simulink model "KneeReflexHuman"  (R2025a)
settings: Solver=ode15s  StartTime=0.0  StopTime=35  FixedStep=0.002  MaxStep=0.001  RelTol=1e-7  AbsTol=1e-9
PreLoadFcn:
  | activationTime=0.01;
  | deactivationTime=0.04;
  | sensoryPulse=2;
  | tapTorque=0;
  | eventTime=20;
  | pulseDuration=0.03;
  | torqueDuration=0.025;
libraries: SNS_Library x16
Description:
  | GUI-built Ia/Ib circuit with two compliant Gait2392 musculotendon blocks and a one-degree-of-freedom knee.
settings Model: Creator=Ben Bolen  LastModifiedBy=Ben Bolen
settings DataIOCC: SignalLogging=off

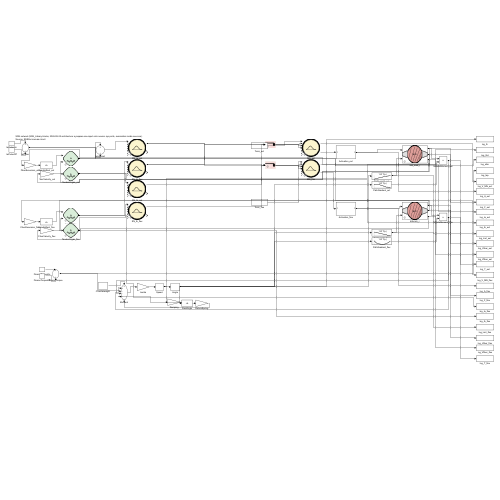
[thumbnail: Simulink's stored preview of the top-level diagram]
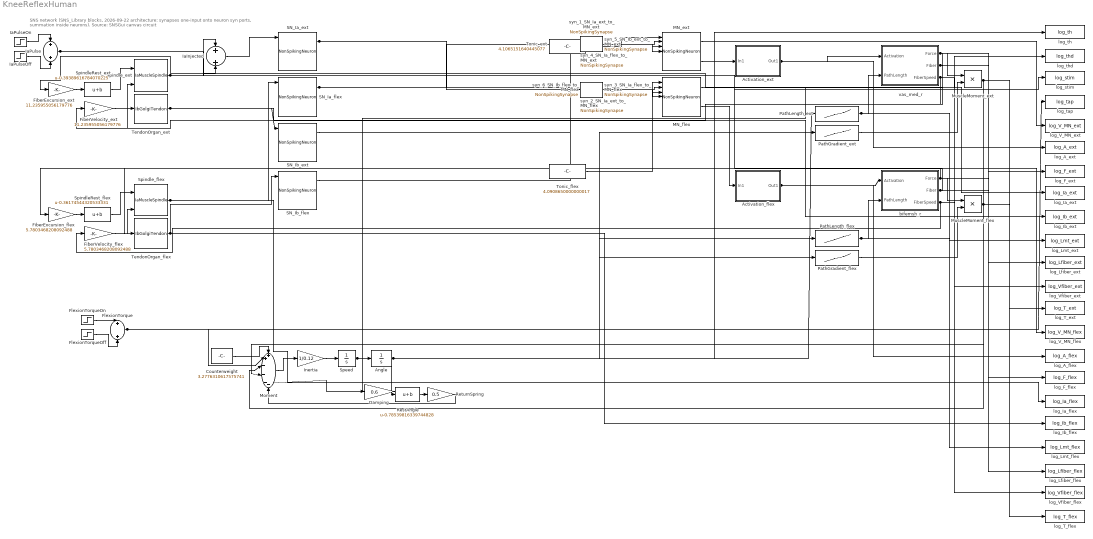
== system KneeReflexHuman ==
  note: SNS network (SNS_Library blocks, 2026-09-22 architecture: synapses one-input onto neuron syn ports, summation inside neurons).
      | Source: SNSGui canvas circuit
  Activation_ext : Subsystem
  Activation_flex : Subsystem
  Angle : Integrator  InitialCondition=0.78539816339744828
  Counterweight : Constant  Value=3.2776310617575741
  Damping : Gain  Gain=0.6
  FiberExcursion_ext : Gain  Gain=11.235955056179776
  FiberExcursion_flex : Gain  Gain=5.7803468208092488
  FiberVelocity_ext : Gain  Gain=11.235955056179776
  FiberVelocity_flex : Gain  Gain=5.7803468208092488
  FlexionTorque : Sum
  FlexionTorqueOff : Step  Time=eventTime+torqueDuration  After=-tapTorque  SampleTime=0
  FlexionTorqueOn : Step  Time=eventTime  After=tapTorque  SampleTime=0
  IaInjected : Sum
  IaPulse : Sum
  IaPulseOff : Step  Time=eventTime+pulseDuration  After=-sensoryPulse  SampleTime=0
  IaPulseOn : Step  Time=eventTime  After=sensoryPulse  SampleTime=0
  Inertia : Gain  Gain=1/0.12
  MN_ext : SNS_Library/NonSpikingNeuron  Vrest=-52  Gm=0.5  Cm=2.5  Thr=-45  Slope=10
  MN_flex : SNS_Library/NonSpikingNeuron  Vrest=-52  Gm=0.5  Cm=2.5  Thr=-45  Slope=10
  Moment : Sum  Inputs=++----
  MuscleMoment_ext : Product
  MuscleMoment_flex : Product
  PathGradient_ext : Lookup_n-D  NumberOfTableDimensions=1  BreakpointsForDimension1=[0 0.017453292519943295 0.034906585039886591 0.05235987755982989 0.069813170079773182 0.087266462599716474 0.10471975511965978 0.12217304763960307 0.13962634015954636 0.15707963267948966 0.17453292519943295 0.19198621771937624 0.20943951023931956 0.22689280275926285 0.24434609527920614 0.26179938779914941 0.27925268031909273 0.29670597283903605 0.31415926535897931 0.33161255787892263 0.3490658503988659 0.36651914291880922 0.38397243543875248 0.4014257279586958 0.41887902047863912 0.43633231299858238 0.4537856055185257 0.47123889803846897 0.48869219055841229 0.50614548307835561 0.52359877559829882 0.54105206811824214 0.55850536063818546 0.57595865315812877 0.59341194567807209 0.6108652381980153 0.62831853071795862 0.64577182323790194 0.66322511575784526 0.68067840827778847 0.69813170079773179 0.71558499331767511 0.73303828583761843 0.75049157835756175 0.76794487087750496 0.78539816339744828 0.8028514559173916 0.82030474843733492 0.83775804095727824 0.85521133347722145 0.87266462599716477 0.89011791851710809 0.90757121103705141 0.92502450355699462 0.94247779607693793 0.95993108859688125 0.97738438111682457 0.99483767363676789 1.0122909661567112 1.0297442586766545 1.0471975511965976 1.064650843716541 1.0821041362364843 1.0995574287564276 1.1170107212763709 1.1344640137963142 1.1519173063162575 1.1693705988362009 1.1868238913561442 1.2042771838760873 1.2217304763960306 1.2391837689159739 1.2566370614359172 1.2740903539558606 1.2915436464758039 1.3089969389957472 1.3264502315156905 1.3439035240356338 1.3613568165555769 1.3788101090755203 1.3962634015954636 1.4137166941154069 1.4311699866353502 1.4486232791552935 1.4660765716752369 1.4835298641951802 1.5009831567151235 1.5184364492350666 1.5358897417550099 1.5533430342749532 1.5707963267948966 1.5882496193148399 1.6057029118347832 1.6231562043547265 1.6406094968746698 1.6580627893946132]  Table=[0.046300541412696045 0.045945528146783335 0.04560618003400034 0.045291206631057568 0.045009747559742942 0.044771407689989967 0.044586287794695818 0.044465010200429353 0.044418738866694063 0.044459193231872661 0.044598655069569046 0.044792320710674169 0.044983515402986986 0.045166436487388571 0.045334488498150194 0.045480452453573142 0.045596644811568894 0.045675065799738478 0.045707536845315852 0.045685826873795007 0.045601767312865145 0.045488375392619018 0.0453804190740692 0.045272500382524589 0.045159280213405172 0.045035490671118006 0.044895946644946429 0.044735556564090159 0.04454933228582144 0.044332398083007075 0.044079998709690885 0.043802898012431105 0.043528262733400512 0.043256947497619311 0.042989173348334131 0.042725127360683068 0.042464964587145354 0.042208809868987306 0.041956759522132597 0.041708882905415239 0.041465223878729411 0.041220522162316059 0.040969567687275568 0.040712466844097947 0.040449332738228566 0.040180285292503316 0.039905451341858217 0.03962496472037294 0.039338966340718776 0.039047604266089025 0.038751033774698324 0.038449417416943923 0.038142925065329424 0.037831733957256544 0.037516028730797221 0.037196001453562624 0.036871851644790808 0.036543786290779014 0.036212019853789669 0.035876774274563865 0.035538278968577371 0.035198023590642488 0.034856945478862256 0.03451445183466019 0.034169952982176559 0.033822863200327721 0.033472601534141611 0.033118592585048387 0.032760267279801386 0.032397063617736394 0.032508073283476019 0.03247750725997104 0.032431791921784733 0.032371807186272486 0.032298273574261599 0.032211774977847177 0.032112778002968467 0.032001648442081303 0.031878665337946643 0.031744033021439806 0.031597891441606234 0.031437980227015702 0.0312622575156037 0.03107113358259856 0.030865597976765073 0.030649752356107715 0.030424658097017637 0.030190733110557224 0.02994839217600519 0.029698048006726905 0.029440112215267402 0.02917504524279816 0.028903309559376068 0.02862532065204686 0.028341496120541262 0.028052256309455396]  ExtrapMethod=Clip  InternalRulePriority=Speed  RndMeth=Simplest
  PathGradient_flex : Lookup_n-D  NumberOfTableDimensions=1  BreakpointsForDimension1=[0 0.017453292519943295 0.034906585039886591 0.05235987755982989 0.069813170079773182 0.087266462599716474 0.10471975511965978 0.12217304763960307 0.13962634015954636 0.15707963267948966 0.17453292519943295 0.19198621771937624 0.20943951023931956 0.22689280275926285 0.24434609527920614 0.26179938779914941 0.27925268031909273 0.29670597283903605 0.31415926535897931 0.33161255787892263 0.3490658503988659 0.36651914291880922 0.38397243543875248 0.4014257279586958 0.41887902047863912 0.43633231299858238 0.4537856055185257 0.47123889803846897 0.48869219055841229 0.50614548307835561 0.52359877559829882 0.54105206811824214 0.55850536063818546 0.57595865315812877 0.59341194567807209 0.6108652381980153 0.62831853071795862 0.64577182323790194 0.66322511575784526 0.68067840827778847 0.69813170079773179 0.71558499331767511 0.73303828583761843 0.75049157835756175 0.76794487087750496 0.78539816339744828 0.8028514559173916 0.82030474843733492 0.83775804095727824 0.85521133347722145 0.87266462599716477 0.89011791851710809 0.90757121103705141 0.92502450355699462 0.94247779607693793 0.95993108859688125 0.97738438111682457 0.99483767363676789 1.0122909661567112 1.0297442586766545 1.0471975511965976 1.064650843716541 1.0821041362364843 1.0995574287564276 1.1170107212763709 1.1344640137963142 1.1519173063162575 1.1693705988362009 1.1868238913561442 1.2042771838760873 1.2217304763960306 1.2391837689159739 1.2566370614359172 1.2740903539558606 1.2915436464758039 1.3089969389957472 1.3264502315156905 1.3439035240356338 1.3613568165555769 1.3788101090755203 1.3962634015954636 1.4137166941154069 1.4311699866353502 1.4486232791552935 1.4660765716752369 1.4835298641951802 1.5009831567151235 1.5184364492350666 1.5358897417550099 1.5533430342749532 1.5707963267948966 1.5882496193148399 1.6057029118347832 1.6231562043547265 1.6406094968746698 1.6580627893946132]  Table=[-0.020361084177321076 -0.02095432404287479 -0.021549948921287549 -0.022147893095183287 -0.022748075168790793 -0.023350397436992496 -0.023954745240616474 -0.024560986306975025 -0.025168970074611902 -0.025778527001181786 -0.026389467853347018 -0.026982156148773202 -0.027536386273640853 -0.028051147190922037 -0.028525485798045501 -0.028958501691153819 -0.029349341935763336 -0.029697195830473311 -0.030001289651172786 -0.030260881364096957 -0.030475255297092951 -0.030664144688230695 -0.030847730623721023 -0.031025982895034908 -0.031198868501991071 -0.031366351184743187 -0.031528390956651269 -0.031684943638144211 -0.031835960391693049 -0.031981387258029709 -0.032121164693761924 -0.032256849277144638 -0.032389988665417535 -0.032520500263503734 -0.032648294373979259 -0.032773273788839895 -0.032895333384571582 -0.033014359720642698 -0.033130230641547929 -0.033242814882547378 -0.033351971679259733 -0.033454060268764241 -0.0335453780438374 -0.033625689200947703 -0.03369476437945839 -0.033752380839864864 -0.033798322644897988 -0.033832380843261095 -0.033854353655739702 -0.033864046663389394 -0.033861272997474864 -0.03384585353079772 -0.03381761707001435 -0.033776400548507925 -0.033722049219339842 -0.033654416847766454 -0.033573365902766245 -0.033478767746981518 -0.033370502824436502 -0.033248460845351928 -0.033112540967333001 -0.032964251381959922 -0.03280509758262215 -0.032634983282771958 -0.032453816040338403 -0.032261507468146849 -0.032057973449924421 -0.031843134361701053 -0.031616915298350867 -0.031379246304984704 -0.031130062612869103 -0.030869260033517858 -0.030596740000038217 -0.030312454668946529 -0.03001636235322382 -0.029708427774943754 -0.029388622319715819 -0.029056924292337999 -0.028713319173009077 -0.028357799873408199 -0.027990366991891596 -0.027610663596923598 -0.027218353429907374 -0.026813481200552089 -0.026396101945645355 -0.025966281237410075 -0.025524095380485421 -0.025069631596368751 -0.024602988194139034 -0.02412427472627245 -0.023633612128355436 -0.0231311328415033 -0.022616980916300468 -0.022091312097095219 -0.021554293885504384 -0.021006105582016245]  ExtrapMethod=Clip  InternalRulePriority=Speed  RndMeth=Simplest
  PathLength_ext : Lookup_n-D  NumberOfTableDimensions=1  BreakpointsForDimension1=[0 0.017453292519943295 0.034906585039886591 0.05235987755982989 0.069813170079773182 0.087266462599716474 0.10471975511965978 0.12217304763960307 0.13962634015954636 0.15707963267948966 0.17453292519943295 0.19198621771937624 0.20943951023931956 0.22689280275926285 0.24434609527920614 0.26179938779914941 0.27925268031909273 0.29670597283903605 0.31415926535897931 0.33161255787892263 0.3490658503988659 0.36651914291880922 0.38397243543875248 0.4014257279586958 0.41887902047863912 0.43633231299858238 0.4537856055185257 0.47123889803846897 0.48869219055841229 0.50614548307835561 0.52359877559829882 0.54105206811824214 0.55850536063818546 0.57595865315812877 0.59341194567807209 0.6108652381980153 0.62831853071795862 0.64577182323790194 0.66322511575784526 0.68067840827778847 0.69813170079773179 0.71558499331767511 0.73303828583761843 0.75049157835756175 0.76794487087750496 0.78539816339744828 0.8028514559173916 0.82030474843733492 0.83775804095727824 0.85521133347722145 0.87266462599716477 0.89011791851710809 0.90757121103705141 0.92502450355699462 0.94247779607693793 0.95993108859688125 0.97738438111682457 0.99483767363676789 1.0122909661567112 1.0297442586766545 1.0471975511965976 1.064650843716541 1.0821041362364843 1.0995574287564276 1.1170107212763709 1.1344640137963142 1.1519173063162575 1.1693705988362009 1.1868238913561442 1.2042771838760873 1.2217304763960306 1.2391837689159739 1.2566370614359172 1.2740903539558606 1.2915436464758039 1.3089969389957472 1.3264502315156905 1.3439035240356338 1.3613568165555769 1.3788101090755203 1.3962634015954636 1.4137166941154069 1.4311699866353502 1.4486232791552935 1.4660765716752369 1.4835298641951802 1.5009831567151235 1.5184364492350666 1.5358897417550099 1.5533430342749532 1.5707963267948966 1.5882496193148399 1.6057029118347832 1.6231562043547265 1.6406094968746698 1.6580627893946132]  Table=[0.17226414023457803 0.17306912241670788 0.1738680327803396 0.17466122014122692 0.17544918902431589 0.17623260748310754 0.17701231549419177 0.17778933384389753 0.17856487341490523 0.17934034476994465 0.18011736791732169 0.18089745113888928 0.18168090068224443 0.18246762406431039 0.1832574203543533 0.18404996782905858 0.18484481449251688 0.18564137127820163 0.18643890774504843 0.18723655007529266 0.18803328117824838 0.18882818077722996 0.18962115663636275 0.19041225644225723 0.19120143416436042 0.19198855119117289 0.1927733776752531 0.19355559407317263 0.19433479286567448 0.19511048044259316 0.19588207913661326 0.19664900249551176 0.19741110599107001 0.19816844482247115 0.19892107891525168 0.19966907175352133 0.20041248980428711 0.20115140197454839 0.20188587909890082 0.202615993455526 0.20334181830858139 0.20406339673360424 0.20478064959247261 0.20549346867270485 0.2062017476771279 0.20690538234198108 0.20760427055673913 0.20829831248552194 0.20898741068995724 0.20967147025336369 0.2103503989061245 0.211024107152123 0.21169250839611231 0.21235551907189359 0.21301305877118049 0.21366505037302669 0.21431142017369864 0.21495209801687493 0.21558701742405872 0.21621611572508853 0.21683933418863893 0.21745662564317342 0.21806797220542951 0.21867335433892215 0.2192727421869049 0.21986609563416265 0.2204533643831465 0.22103448804408499 0.22160939623870357 0.22217800871717458 0.22274598949535074 0.22331311842427704 0.22387958026527199 0.22444511854181917 0.22500949070796325 0.22557246557043772 0.22613382107738966 0.22669334241891756 0.22725082039347982 0.22780605000157636 0.22835882923420606 0.22890894429032693 0.22945612978007696 0.2300001133427981 0.23054063134628333 0.2310774678055289 0.2316104557277896 0.23213943734621723 0.23266426215892685 0.23318478688379607 0.23370087543096607 0.23421239917621736 0.23471923783150911 0.23522127862909314 0.23571841607032532 0.23621055196811466]  ExtrapMethod=Clip  InternalRulePriority=Speed  RndMeth=Simplest
  PathLength_flex : Lookup_n-D  NumberOfTableDimensions=1  BreakpointsForDimension1=[0 0.017453292519943295 0.034906585039886591 0.05235987755982989 0.069813170079773182 0.087266462599716474 0.10471975511965978 0.12217304763960307 0.13962634015954636 0.15707963267948966 0.17453292519943295 0.19198621771937624 0.20943951023931956 0.22689280275926285 0.24434609527920614 0.26179938779914941 0.27925268031909273 0.29670597283903605 0.31415926535897931 0.33161255787892263 0.3490658503988659 0.36651914291880922 0.38397243543875248 0.4014257279586958 0.41887902047863912 0.43633231299858238 0.4537856055185257 0.47123889803846897 0.48869219055841229 0.50614548307835561 0.52359877559829882 0.54105206811824214 0.55850536063818546 0.57595865315812877 0.59341194567807209 0.6108652381980153 0.62831853071795862 0.64577182323790194 0.66322511575784526 0.68067840827778847 0.69813170079773179 0.71558499331767511 0.73303828583761843 0.75049157835756175 0.76794487087750496 0.78539816339744828 0.8028514559173916 0.82030474843733492 0.83775804095727824 0.85521133347722145 0.87266462599716477 0.89011791851710809 0.90757121103705141 0.92502450355699462 0.94247779607693793 0.95993108859688125 0.97738438111682457 0.99483767363676789 1.0122909661567112 1.0297442586766545 1.0471975511965976 1.064650843716541 1.0821041362364843 1.0995574287564276 1.1170107212763709 1.1344640137963142 1.1519173063162575 1.1693705988362009 1.1868238913561442 1.2042771838760873 1.2217304763960306 1.2391837689159739 1.2566370614359172 1.2740903539558606 1.2915436464758039 1.3089969389957472 1.3264502315156905 1.3439035240356338 1.3613568165555769 1.3788101090755203 1.3962634015954636 1.4137166941154069 1.4311699866353502 1.4486232791552935 1.4660765716752369 1.4835298641951802 1.5009831567151235 1.5184364492350666 1.5358897417550099 1.5533430342749532 1.5707963267948966 1.5882496193148399 1.6057029118347832 1.6231562043547265 1.6406094968746698 1.6580627893946132]  Table=[0.24625075890103157 0.2458902174580414 0.24551930112851292 0.24513796883726094 0.24474618079199639 0.24434389876245297 0.24393108637064406 0.2435077093925001 0.24307373607115063 0.24262913744213851 0.24217388767086862 0.24170807721638785 0.24123225649552227 0.2407471056410122 0.24025332191832333 0.23975161876020945 0.23924272489258069 0.23872738355168194 0.23820635179281544 0.23768039989104867 0.23715031083454793 0.23661676122560141 0.23607996111411669 0.23554000332275599 0.23499698122510049 0.23445098879845916 0.2339021206848379 0.23335047226005468 0.23279613971097904 0.23223922012087819 0.2316798115628457 0.23111800376309391 0.23055384991648156 0.22998739515578978 0.22941868611673941 0.22884777106551743 0.22827470003339995 0.22769952495841272 0.22712229983396864 0.22654308086441877 0.2259619266274511 0.22537891852748476 0.22479422229102369 0.22420802797125947 0.22362052968096371 0.22303192547848766 0.22244241725062483 0.22185221059228996 0.22126151468296998 0.2206705421599082 0.22007950898798781 0.21948863432628821 0.21889814039129254 0.21830825231673309 0.21771919801006898 0.21713120800559954 0.21654451531422519 0.21595935526987822 0.21537596537265757 0.2147945851287113 0.2142154558869237 0.21363881136446372 0.21306484964892342 0.21249376120230673 0.21192573813388765 0.21136097413128307 0.21079966438780465 0.21024200552599301 0.20968819551724283 0.20913843359743051 0.20859292017846437 0.2080518570165715 0.20751544789851614 0.20698389775873763 0.20645741231334186 0.20593619795044979 0.20542046161611893 0.20491041069581317 0.20440625289140499 0.20390819609370497 0.20341644825052965 0.20293121936125627 0.20245272761886318 0.2019811926777286 0.20151683332208922 0.20105986728396449 0.20061051105754235 0.20016897971023481 0.19973548669063176 0.19931024363360408 0.19889346016282591 0.19848534369100729 0.19808609921815051 0.19769592912816084 0.19731503298416755 0.19694360732292446]  ExtrapMethod=Clip  InternalRulePriority=Speed  RndMeth=Simplest
  RestAngle : Bias  Bias=-0.78539816339744828  SaturateOnIntegerOverflow=off
  ReturnSpring : Gain  Gain=0.5
  SN_Ia_ext : SNS_Library/NonSpikingNeuron  Vrest=-52  Gm=0.4  Cm=2  Thr=-55  Slope=1
  SN_Ia_flex : SNS_Library/NonSpikingNeuron  Vrest=-52  Gm=0.4  Cm=2  Thr=-55  Slope=1
  SN_Ib_ext : SNS_Library/NonSpikingNeuron  Vrest=-52  Gm=0.4  Cm=2  Thr=-55  Slope=1
  SN_Ib_flex : SNS_Library/NonSpikingNeuron  Vrest=-52  Gm=0.4  Cm=2  Thr=-55  Slope=1
  Speed : Integrator
  SpindleRest_ext : Bias  Bias=-0.39389616784070225  SaturateOnIntegerOverflow=off
  SpindleRest_flex : Bias  Bias=-0.36174544320533331  SaturateOnIntegerOverflow=off
  Spindle_ext : SNS_Library/IaMuscleSpindle  Imax=10  Wl=6  Wv=3
  Spindle_flex : SNS_Library/IaMuscleSpindle  Imax=10  Wl=6  Wv=3
  TendonOrgan_ext : SNS_Library/IbGolgiTendon  Imax=10  Kf=0.02
  TendonOrgan_flex : SNS_Library/IbGolgiTendon  Imax=10  Kf=0.022200000000000001
  Tonic_ext : Constant  Value=4.1065151640445077
  Tonic_flex : Constant  Value=4.0908650000000017
  bifemsh_r : Subsystem  mask(Gait2392 Thelen2003 biological muscle){}
      mask help: Elastic tendon, active and passive fibers, and constant-height pennation driven by Gait2392 parameters.
      mask Display:
      | patch([-0.58 -0.5558 -0.5317 -0.5075 -0.4833 -0.4592 -0.435 -0.4108 -0.3867 -0.3625 -0.3383 -0.3142 -0.29 -0.2658 -0.2417 -0.2175 -0.1933 -0.1692 -0.145 -0.1208 -0.09667 -0.0725 -0.04833 -0.02417 0 0.02417 0.04833 0.0725 0.09667 0.1208 0.145 0.1692 0.1933 0.2175 0.2417 0.2658 0.29 0.3142 0.3383 0.3625 0.3867 0.4108 0.435 0.4592 0.4833 0.5075 0.5317 0.5558 0.58 0.58 0.5558 0.5317 0.5075 0.4833 0.4592 0.435 0.4108 0.3867 0.3625 0.3383 0.3142 0.29 0.2658 0.2417 0.2175 0.1933 0.1692 0.145 0.1208 0.09667 0.0725 0.04833 0.02417 0 -0.02417 -0.04833 -0.0725 -0.09667 -0.1208 -0.145 -0.1692 -0.1933 -0.2175 -0.2417 -0.2658 -0.29 -0.3142 -0.3383 -0.3625 -0.3867 -0.4108 -0.435 -0.4592 -0.4833 -0.5075 -0.5317 -0.5558 -0.58], [0.022 0.07714 0.1114 0.1399 0.1647 0.1868 0.2067 0.2249 0.2414 0.2565 0.2703 0.2829 0.2943 0.3047 0.314 0.3224 0.3298 0.3362 0.3418 0.3465 0.3503 0.3532 0.3553 0.3566 0.357 0.3566 0.3553 0.3532 0.3503 0.3465 0.3418 0.3362 0.3298 0.3224 0.314 0.3047 0.2943 0.2829 0.2703 0.2565 0.2414 0.2249 0.2067 0.1868 0.1647 0.1399 0.1114 0.07714 0.022 0.022 -0.07714 -0.1114 -0.1399 -0.1647 -0.1868 -0.2067 -0.2249 -0.2414 -0.2565 -0.2703 -0.2829 -0.2943 -0.3047 -0.314 -0.3224 -0.3298 -0.3362 -0.3418 -0.3465 -0.3503 -0.3532 -0.3553 -0.3566 -0.357 -0.3566 -0.3553 -0.3532 -0.3503 -0.3465 -0.3418 -0.3362 -0.3298 -0.3224 -0.314 -0.3047 -0.2943 -0.2829 -0.2703 -0.2565 -0.2414 -0.2249 -0.2067 -0.1868 -0.1647 -0.1399 -0.1114 -0.07714 0.022], [0 0 0]);
      | patch([-0.58 -0.5558 -0.5317 -0.5075 -0.4833 -0.4592 -0.435 -0.4108 -0.3867 -0.3625 -0.3383 -0.3142 -0.29 -0.2658 -0.2417 -0.2175 -0.1933 -0.1692 -0.145 -0.1208 -0.09667 -0.0725 -0.04833 -0.02417 0 0.02417 0.04833 0.0725 0.09667 0.1208 0.145 0.1692 0.1933 0.2175 0.2417 0.2658 0.29 0.3142 0.3383 0.3625 0.3867 0.4108 0.435 0.4592 0.4833 0.5075 0.5317 0.5558 0.58 0.58 0.5558 0.5317 0.5075 0.4833 0.4592 0.435 0.4108 0.3867 0.3625 0.3383 0.3142 0.29 0.2658 0.2417 0.2175 0.1933 0.1692 0.145 0.1208 0.09667 0.0725 0.04833 0.02417 0 -0.02417 -0.04833 -0.0725 -0.09667 -0.1208 -0.145 -0.1692 -0.1933 -0.2175 -0.2417 -0.2658 -0.29 -0.3142 -0.3383 -0.3625 -0.3867 -0.4108 -0.435 -0.4592 -0.4833 -0.5075 -0.5317 -0.5558 -0.58], [0 0.05514 0.08943 0.1179 0.1427 0.1648 0.1847 0.2029 0.2194 0.2345 0.2483 0.2609 0.2723 0.2827 0.292 0.3004 0.3078 0.3142 0.3198 0.3245 0.3283 0.3312 0.3333 0.3346 0.335 0.3346 0.3333 0.3312 0.3283 0.3245 0.3198 0.3142 0.3078 0.3004 0.292 0.2827 0.2723 0.2609 0.2483 0.2345 0.2194 0.2029 0.1847 0.1648 0.1427 0.1179 0.08943 0.05514 0 -0 -0.05514 -0.08943 -0.1179 -0.1427 -0.1648 -0.1847 -0.2029 -0.2194 -0.2345 -0.2483 -0.2609 -0.2723 -0.2827 -0.292 -0.3004 -0.3078 -0.3142 -0.3198 -0.3245 -0.3283 -0.3312 -0.3333 -0.3346 -0.335 -0.3346 -0.3333 -0.3312 -0.3283 -0.3245 -0.3198 -0.3142 -0.3078 -0.3004 -0.292 -0.2827 -0.2723 -0.2609 -0.2483 -0.2345 -0.2194 -0.2029 -0.1847 -0.1648 -0.1427 -0.1179 -0.08943 -0.05514 -0], [0.87 0.62 0.6]);
      | color('black');
      | plot([-0.46 -0.2855], [-0.1476 0.2469]);
      | plot([-0.305 -0.02282], [-0.2388 0.3012]);
      | plot([-0.15 0.1889], [-0.2868 0.2781]);
      | plot([0.005 0.3612], [-0.3015 0.2117]);
      | plot([0.16 0.4965], [-0.2848 0.1166]);
      | plot([0.315 0.52], [-0.2344 0.09333]);
      | plot([0.47 0.52], [-0.1396 0.09333]);
      | patch([0.58 0.95 0.95 0.58], [-0.148 -0.068 0.068 0.148], [0 0 0]);
      | patch([0.58 0.95 0.95 0.58], [-0.13 -0.05 0.05 0.13], [0.88 0.88 0.88]);
      | patch([-0.58 -0.95 -0.95 -0.58], [-0.148 -0.068 0.068 0.148], [0 0 0]);
      | patch([-0.58 -0.95 -0.95 -0.58], [-0.13 -0.05 0.05 0.13], [0.88 0.88 0.88]);
      | disp('BIO');
  log_A_ext : ToWorkspace  VariableName=log_A_ext  SaveFormat=Timeseries  SampleTime=-1
  log_A_flex : ToWorkspace  VariableName=log_A_flex  SaveFormat=Timeseries  SampleTime=-1
  log_F_ext : ToWorkspace  VariableName=log_F_ext  SaveFormat=Timeseries  SampleTime=-1
  log_F_flex : ToWorkspace  VariableName=log_F_flex  SaveFormat=Timeseries  SampleTime=-1
  log_Ia_ext : ToWorkspace  VariableName=log_Ia_ext  SaveFormat=Timeseries  SampleTime=-1
  log_Ia_flex : ToWorkspace  VariableName=log_Ia_flex  SaveFormat=Timeseries  SampleTime=-1
  log_Ib_ext : ToWorkspace  VariableName=log_Ib_ext  SaveFormat=Timeseries  SampleTime=-1
  log_Ib_flex : ToWorkspace  VariableName=log_Ib_flex  SaveFormat=Timeseries  SampleTime=-1
  log_Lfiber_ext : ToWorkspace  VariableName=log_Lfiber_ext  SaveFormat=Timeseries  SampleTime=-1
  log_Lfiber_flex : ToWorkspace  VariableName=log_Lfiber_flex  SaveFormat=Timeseries  SampleTime=-1
  log_Lmt_ext : ToWorkspace  VariableName=log_Lmt_ext  SaveFormat=Timeseries  SampleTime=-1
  log_Lmt_flex : ToWorkspace  VariableName=log_Lmt_flex  SaveFormat=Timeseries  SampleTime=-1
  log_T_ext : ToWorkspace  VariableName=log_T_ext  SaveFormat=Timeseries  SampleTime=-1
  log_T_flex : ToWorkspace  VariableName=log_T_flex  SaveFormat=Timeseries  SampleTime=-1
  log_V_MN_ext : ToWorkspace  VariableName=log_V_MN_ext  SaveFormat=Timeseries  SampleTime=-1
  log_V_MN_flex : ToWorkspace  VariableName=log_V_MN_flex  SaveFormat=Timeseries  SampleTime=-1
  log_Vfiber_ext : ToWorkspace  VariableName=log_Vfiber_ext  SaveFormat=Timeseries  SampleTime=-1
  log_Vfiber_flex : ToWorkspace  VariableName=log_Vfiber_flex  SaveFormat=Timeseries  SampleTime=-1
  log_stim : ToWorkspace  VariableName=log_stim  SaveFormat=Timeseries  SampleTime=-1
  log_tap : ToWorkspace  VariableName=log_tap  SaveFormat=Timeseries  SampleTime=-1
  log_th : ToWorkspace  VariableName=log_th  SaveFormat=Timeseries  SampleTime=-1
  log_thd : ToWorkspace  VariableName=log_thd  SaveFormat=Timeseries  SampleTime=-1
  syn_1_SN_Ia_ext_to_MN_ext : SNS_Library/NonSpikingSynapse  gmax=0.009  Esyn=0  ThrPre=-45  SlopePre=10
  syn_2_SN_Ia_ext_to_MN_flex : SNS_Library/NonSpikingSynapse  gmax=0.0075  Esyn=-72  ThrPre=-45  SlopePre=10
  syn_3_SN_Ia_flex_to_MN_flex : SNS_Library/NonSpikingSynapse  gmax=0.009  Esyn=0  ThrPre=-45  SlopePre=10
  syn_4_SN_Ia_flex_to_MN_ext : SNS_Library/NonSpikingSynapse  gmax=0.0075  Esyn=-72  ThrPre=-45  SlopePre=10
  syn_5_SN_Ib_ext_to_MN_ext : SNS_Library/NonSpikingSynapse  gmax=0.01  Esyn=-72  ThrPre=-45  SlopePre=10
  syn_6_SN_Ib_flex_to_MN_flex : SNS_Library/NonSpikingSynapse  gmax=0.01  Esyn=-72  ThrPre=-45  SlopePre=10
  vas_med_r : Subsystem  mask(Gait2392 Thelen2003 biological muscle){}
      mask help: Elastic tendon, active and passive fibers, and constant-height pennation driven by Gait2392 parameters.
      mask Display:
      | patch([-0.58 -0.5558 -0.5317 -0.5075 -0.4833 -0.4592 -0.435 -0.4108 -0.3867 -0.3625 -0.3383 -0.3142 -0.29 -0.2658 -0.2417 -0.2175 -0.1933 -0.1692 -0.145 -0.1208 -0.09667 -0.0725 -0.04833 -0.02417 0 0.02417 0.04833 0.0725 0.09667 0.1208 0.145 0.1692 0.1933 0.2175 0.2417 0.2658 0.29 0.3142 0.3383 0.3625 0.3867 0.4108 0.435 0.4592 0.4833 0.5075 0.5317 0.5558 0.58 0.58 0.5558 0.5317 0.5075 0.4833 0.4592 0.435 0.4108 0.3867 0.3625 0.3383 0.3142 0.29 0.2658 0.2417 0.2175 0.1933 0.1692 0.145 0.1208 0.09667 0.0725 0.04833 0.02417 0 -0.02417 -0.04833 -0.0725 -0.09667 -0.1208 -0.145 -0.1692 -0.1933 -0.2175 -0.2417 -0.2658 -0.29 -0.3142 -0.3383 -0.3625 -0.3867 -0.4108 -0.435 -0.4592 -0.4833 -0.5075 -0.5317 -0.5558 -0.58], [0.022 0.07714 0.1114 0.1399 0.1647 0.1868 0.2067 0.2249 0.2414 0.2565 0.2703 0.2829 0.2943 0.3047 0.314 0.3224 0.3298 0.3362 0.3418 0.3465 0.3503 0.3532 0.3553 0.3566 0.357 0.3566 0.3553 0.3532 0.3503 0.3465 0.3418 0.3362 0.3298 0.3224 0.314 0.3047 0.2943 0.2829 0.2703 0.2565 0.2414 0.2249 0.2067 0.1868 0.1647 0.1399 0.1114 0.07714 0.022 0.022 -0.07714 -0.1114 -0.1399 -0.1647 -0.1868 -0.2067 -0.2249 -0.2414 -0.2565 -0.2703 -0.2829 -0.2943 -0.3047 -0.314 -0.3224 -0.3298 -0.3362 -0.3418 -0.3465 -0.3503 -0.3532 -0.3553 -0.3566 -0.357 -0.3566 -0.3553 -0.3532 -0.3503 -0.3465 -0.3418 -0.3362 -0.3298 -0.3224 -0.314 -0.3047 -0.2943 -0.2829 -0.2703 -0.2565 -0.2414 -0.2249 -0.2067 -0.1868 -0.1647 -0.1399 -0.1114 -0.07714 0.022], [0 0 0]);
      | patch([-0.58 -0.5558 -0.5317 -0.5075 -0.4833 -0.4592 -0.435 -0.4108 -0.3867 -0.3625 -0.3383 -0.3142 -0.29 -0.2658 -0.2417 -0.2175 -0.1933 -0.1692 -0.145 -0.1208 -0.09667 -0.0725 -0.04833 -0.02417 0 0.02417 0.04833 0.0725 0.09667 0.1208 0.145 0.1692 0.1933 0.2175 0.2417 0.2658 0.29 0.3142 0.3383 0.3625 0.3867 0.4108 0.435 0.4592 0.4833 0.5075 0.5317 0.5558 0.58 0.58 0.5558 0.5317 0.5075 0.4833 0.4592 0.435 0.4108 0.3867 0.3625 0.3383 0.3142 0.29 0.2658 0.2417 0.2175 0.1933 0.1692 0.145 0.1208 0.09667 0.0725 0.04833 0.02417 0 -0.02417 -0.04833 -0.0725 -0.09667 -0.1208 -0.145 -0.1692 -0.1933 -0.2175 -0.2417 -0.2658 -0.29 -0.3142 -0.3383 -0.3625 -0.3867 -0.4108 -0.435 -0.4592 -0.4833 -0.5075 -0.5317 -0.5558 -0.58], [0 0.05514 0.08943 0.1179 0.1427 0.1648 0.1847 0.2029 0.2194 0.2345 0.2483 0.2609 0.2723 0.2827 0.292 0.3004 0.3078 0.3142 0.3198 0.3245 0.3283 0.3312 0.3333 0.3346 0.335 0.3346 0.3333 0.3312 0.3283 0.3245 0.3198 0.3142 0.3078 0.3004 0.292 0.2827 0.2723 0.2609 0.2483 0.2345 0.2194 0.2029 0.1847 0.1648 0.1427 0.1179 0.08943 0.05514 0 -0 -0.05514 -0.08943 -0.1179 -0.1427 -0.1648 -0.1847 -0.2029 -0.2194 -0.2345 -0.2483 -0.2609 -0.2723 -0.2827 -0.292 -0.3004 -0.3078 -0.3142 -0.3198 -0.3245 -0.3283 -0.3312 -0.3333 -0.3346 -0.335 -0.3346 -0.3333 -0.3312 -0.3283 -0.3245 -0.3198 -0.3142 -0.3078 -0.3004 -0.292 -0.2827 -0.2723 -0.2609 -0.2483 -0.2345 -0.2194 -0.2029 -0.1847 -0.1648 -0.1427 -0.1179 -0.08943 -0.05514 -0], [0.87 0.62 0.6]);
      | color('black');
      | plot([-0.46 -0.2855], [-0.1476 0.2469]);
      | plot([-0.305 -0.02282], [-0.2388 0.3012]);
      | plot([-0.15 0.1889], [-0.2868 0.2781]);
      | plot([0.005 0.3612], [-0.3015 0.2117]);
      | plot([0.16 0.4965], [-0.2848 0.1166]);
      | plot([0.315 0.52], [-0.2344 0.09333]);
      | plot([0.47 0.52], [-0.1396 0.09333]);
      | patch([0.58 0.95 0.95 0.58], [-0.148 -0.068 0.068 0.148], [0 0 0]);
      | patch([0.58 0.95 0.95 0.58], [-0.13 -0.05 0.05 0.13], [0.88 0.88 0.88]);
      | patch([-0.58 -0.95 -0.95 -0.58], [-0.148 -0.068 0.068 0.148], [0 0 0]);
      | patch([-0.58 -0.95 -0.95 -0.58], [-0.13 -0.05 0.05 0.13], [0.88 0.88 0.88]);
      | disp('BIO');
  wires:
  syn_1_SN_Ia_ext_to_MN_ext/1 -> MN_ext/2
  syn_4_SN_Ia_flex_to_MN_ext/1 -> MN_ext/3
  syn_5_SN_Ib_ext_to_MN_ext/1 -> MN_ext/4
  syn_2_SN_Ia_ext_to_MN_flex/1 -> MN_flex/2
  syn_3_SN_Ia_flex_to_MN_flex/1 -> MN_flex/3
  syn_6_SN_Ib_flex_to_MN_flex/1 -> MN_flex/4
  SN_Ia_ext/1 -> syn_1_SN_Ia_ext_to_MN_ext/1, syn_2_SN_Ia_ext_to_MN_flex/1
  SN_Ia_flex/1 -> syn_3_SN_Ia_flex_to_MN_flex/1, syn_4_SN_Ia_flex_to_MN_ext/1
  SN_Ib_ext/1 -> syn_5_SN_Ib_ext_to_MN_ext/1
  SN_Ib_flex/1 -> syn_6_SN_Ib_flex_to_MN_flex/1
  Moment/1 -> Inertia/1
  Inertia/1 -> Speed/1
  Speed/1 -> Angle/1, Damping/1, log_thd/1
  Angle/1 -> RestAngle/1, PathLength_ext/1, PathGradient_ext/1, PathLength_flex/1, PathGradient_flex/1, log_th/1
  RestAngle/1 -> ReturnSpring/1
  Counterweight/1 -> Moment/1
  Damping/1 -> Moment/5
  ReturnSpring/1 -> Moment/6
  IaPulseOn/1 -> IaPulse/1
  IaPulseOff/1 -> IaPulse/2
  FlexionTorqueOn/1 -> FlexionTorque/1
  FlexionTorqueOff/1 -> FlexionTorque/2
  FlexionTorque/1 -> Moment/2, log_tap/1
  MN_ext/2 -> Activation_ext/1(In1)
  Activation_ext/1(Out1) -> vas_med_r/1(Activation), log_A_ext/1
  PathLength_ext/1 -> vas_med_r/2(PathLength), log_Lmt_ext/1
  vas_med_r/1(Force) -> MuscleMoment_ext/1, TendonOrgan_ext/1, log_F_ext/1
  PathGradient_ext/1 -> MuscleMoment_ext/2
  MuscleMoment_ext/1 -> Moment/3, log_T_ext/1
  vas_med_r/2(Fiber) -> FiberExcursion_ext/1, log_Lfiber_ext/1
  FiberExcursion_ext/1 -> SpindleRest_ext/1
  vas_med_r/3(FiberSpeed) -> FiberVelocity_ext/1, log_Vfiber_ext/1
  SpindleRest_ext/1 -> Spindle_ext/1
  FiberVelocity_ext/1 -> Spindle_ext/2
  Spindle_ext/1 -> IaInjected/1, log_Ia_ext/1
  IaPulse/1 -> IaInjected/2, log_stim/1
  IaInjected/1 -> SN_Ia_ext/1
  TendonOrgan_ext/1 -> SN_Ib_ext/1, log_Ib_ext/1
  Tonic_ext/1 -> MN_ext/1
  MN_flex/2 -> Activation_flex/1(In1)
  Activation_flex/1(Out1) -> bifemsh_r/1(Activation), log_A_flex/1
  PathLength_flex/1 -> bifemsh_r/2(PathLength), log_Lmt_flex/1
  bifemsh_r/1(Force) -> MuscleMoment_flex/1, TendonOrgan_flex/1, log_F_flex/1
  PathGradient_flex/1 -> MuscleMoment_flex/2
  MuscleMoment_flex/1 -> Moment/4, log_T_flex/1
  bifemsh_r/2(Fiber) -> FiberExcursion_flex/1, log_Lfiber_flex/1
  FiberExcursion_flex/1 -> SpindleRest_flex/1
  bifemsh_r/3(FiberSpeed) -> FiberVelocity_flex/1, log_Vfiber_flex/1
  SpindleRest_flex/1 -> Spindle_flex/1
  FiberVelocity_flex/1 -> Spindle_flex/2
  Spindle_flex/1 -> SN_Ia_flex/1, log_Ia_flex/1
  TendonOrgan_flex/1 -> SN_Ib_flex/1, log_Ib_flex/1
  Tonic_flex/1 -> MN_flex/1
  MN_ext/1 -> log_V_MN_ext/1
  MN_flex/1 -> log_V_MN_flex/1

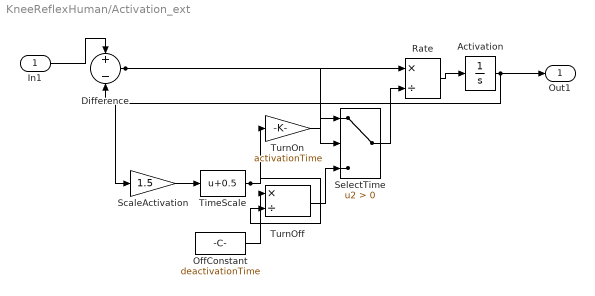
== system KneeReflexHuman/Activation_ext ==
  In1 : Inport
  Activation : Integrator  InitialCondition=0.12  LimitOutput=on  UpperSaturationLimit=1  LowerSaturationLimit=0.01
  Difference : Sum  Inputs=+-
  OffConstant : Constant  Value=deactivationTime
  Rate : Product  Inputs=*/
  ScaleActivation : Gain  Gain=1.5
  SelectTime : Switch  Criteria=u2 > Threshold  SaturateOnIntegerOverflow=off  InputSameDT=off
  TimeScale : Bias  Bias=0.5  SaturateOnIntegerOverflow=off
  TurnOff : Product  Inputs=*/
  TurnOn : Gain  Gain=activationTime
  Out1 : Outport
  wires:
  In1/1 -> Difference/1
  Activation/1 -> Difference/2, ScaleActivation/1, Out1/1
  ScaleActivation/1 -> TimeScale/1
  TimeScale/1 -> TurnOn/1, TurnOff/2
  OffConstant/1 -> TurnOff/1
  TurnOn/1 -> SelectTime/1
  Difference/1 -> SelectTime/2, Rate/1
  TurnOff/1 -> SelectTime/3
  SelectTime/1 -> Rate/2
  Rate/1 -> Activation/1

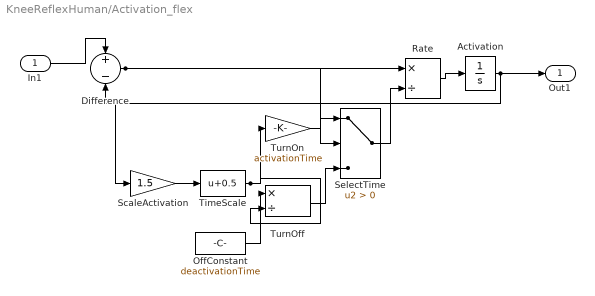
== system KneeReflexHuman/Activation_flex ==
  In1 : Inport
  Activation : Integrator  InitialCondition=0.12  LimitOutput=on  UpperSaturationLimit=1  LowerSaturationLimit=0.01
  Difference : Sum  Inputs=+-
  OffConstant : Constant  Value=deactivationTime
  Rate : Product  Inputs=*/
  ScaleActivation : Gain  Gain=1.5
  SelectTime : Switch  Criteria=u2 > Threshold  SaturateOnIntegerOverflow=off  InputSameDT=off
  TimeScale : Bias  Bias=0.5  SaturateOnIntegerOverflow=off
  TurnOff : Product  Inputs=*/
  TurnOn : Gain  Gain=activationTime
  Out1 : Outport
  wires:
  In1/1 -> Difference/1
  Activation/1 -> Difference/2, ScaleActivation/1, Out1/1
  ScaleActivation/1 -> TimeScale/1
  TimeScale/1 -> TurnOn/1, TurnOff/2
  OffConstant/1 -> TurnOff/1
  TurnOn/1 -> SelectTime/1
  Difference/1 -> SelectTime/2, Rate/1
  TurnOff/1 -> SelectTime/3
  SelectTime/1 -> Rate/2
  Rate/1 -> Activation/1

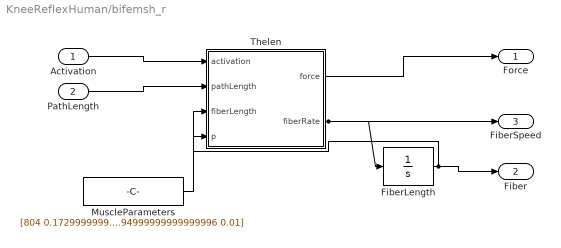
== system KneeReflexHuman/bifemsh_r ==
  Activation : Inport
  PathLength : Inport  Port=2
  FiberLength : Integrator  InitialCondition=0.14908196167452265  LimitOutput=on  LowerSaturationLimit=0.067937024160108245
  MuscleParameters : Constant  Value=[804 0.17299999999999999 0.088999999999999996 0.40142573000000004 10 0.033000000000000002 0.59999999999999998 4 0.5 0.29999999999999999 1.8 0.94999999999999996 0.01]
  Thelen : MATLAB Function  TreatAsAtomicUnit=on
  Force : Outport
  Fiber : Outport  Port=2
  FiberSpeed : Outport  Port=3
  wires:
  Activation/1 -> Thelen/1(activation)
  PathLength/1 -> Thelen/2(pathLength)
  FiberLength/1 -> Thelen/3(fiberLength), Fiber/1
  MuscleParameters/1 -> Thelen/4(p)
  Thelen/1(force) -> Force/1
  Thelen/2(fiberRate) -> FiberLength/1, FiberSpeed/1

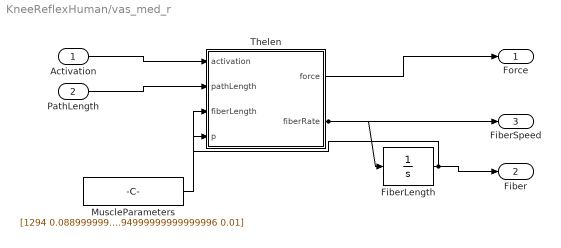
== system KneeReflexHuman/vas_med_r ==
  Activation : Inport
  PathLength : Inport  Port=2
  FiberLength : Integrator  InitialCondition=0.079556758937822492  LimitOutput=on  LowerSaturationLimit=0.0077959385061221222
  MuscleParameters : Constant  Value=[1294 0.088999999999999996 0.126 0.087266460000000004 10 0.033000000000000002 0.59999999999999998 4 0.5 0.29999999999999999 1.8 0.94999999999999996 0.01]
  Thelen : MATLAB Function  TreatAsAtomicUnit=on
  Force : Outport
  Fiber : Outport  Port=2
  FiberSpeed : Outport  Port=3
  wires:
  Activation/1 -> Thelen/1(activation)
  PathLength/1 -> Thelen/2(pathLength)
  FiberLength/1 -> Thelen/3(fiberLength), Fiber/1
  MuscleParameters/1 -> Thelen/4(p)
  Thelen/1(force) -> Force/1
  Thelen/2(fiberRate) -> FiberLength/1, FiberSpeed/1

== matlab function KneeReflexHuman/bifemsh_r/Thelen ==
  data: activation input; force output; pathLength input; fiberLength input; p input; fiberRate output
function [force, fiberRate] = thelen_reflex_fiber(activation, pathLength, fiberLength, p)
% Elastic tendon and fixed-height pennation. Units are N, m, and s.
% OpenSim 4.4 Thelen2003Muscle::calcfse, calcfpe, and calcdlceN.
% p = F0, lopt, lslack, pennation angle (rad), vmax, tendon strain,
% passive strain, passive and active curve shape, Af, Flen, FV extrapolation, amin.
%#codegen
height = p(2)*sin(p(4));
minFiber = max(0.01*p(2),height/sin(acos(0.1)));
fiber = max(minFiber,fiberLength);
projected = sqrt(max(fiber^2-height^2,0));
cosPennation = projected/fiber;
strain = (pathLength-projected)/p(3)-1;
toe = 99*exp(3)/(166*exp(3)-67)*p(6);
if strain <= 0
    tendon = 0;
elseif strain < toe
    tendon = 0.33*expm1(3*strain/toe)/expm1(3);
else
    tendon = 0.33+0.67*(strain-toe)/(p(6)-toe);
end
force = p(1)*tendon;
normalizedLength = fiber/p(2);
activeLength = exp(-(normalizedLength-1)^2/p(9));
passive = expm1(p(8)*max(normalizedLength-1,0)/p(7))/expm1(p(8));
a = min(1,max(p(13),activation));
activeIsometric = a*activeLength;
activeForce = tendon/cosPennation-passive;
% Outside the original concentric/eccentric branches, OpenSim extends
% the tangent from its boundary to keep velocity finite.
threshold = p(12)*p(11)*activeIsometric;
edgeForce = min(threshold,max(0,activeForce));
if edgeForce <= activeIsometric
    denom = activeIsometric+edgeForce/p(10);
    deriv = 1/p(10);
else
    scale = (2+2/p(10))/(p(11)-1);
    denom = scale*(activeIsometric*p(11)-edgeForce);
    deriv = -scale;
end
speedScale = 0.25+0.75*a;
edgeSpeed = speedScale*(edgeForce-activeIsometric)/denom;
slope = (speedScale-edgeSpeed*deriv)/denom;
fiberRate = (edgeSpeed+slope*(activeForce-edgeForce))*p(5)*p(2);
if fiberLength <= minFiber && fiberRate < 0
    fiberRate = 0;
end
end

== matlab function KneeReflexHuman/vas_med_r/Thelen ==
  data: activation input; force output; pathLength input; fiberLength input; p input; fiberRate output
function [force, fiberRate] = thelen_reflex_fiber(activation, pathLength, fiberLength, p)
% Elastic tendon and fixed-height pennation. Units are N, m, and s.
% OpenSim 4.4 Thelen2003Muscle::calcfse, calcfpe, and calcdlceN.
% p = F0, lopt, lslack, pennation angle (rad), vmax, tendon strain,
% passive strain, passive and active curve shape, Af, Flen, FV extrapolation, amin.
%#codegen
height = p(2)*sin(p(4));
minFiber = max(0.01*p(2),height/sin(acos(0.1)));
fiber = max(minFiber,fiberLength);
projected = sqrt(max(fiber^2-height^2,0));
cosPennation = projected/fiber;
strain = (pathLength-projected)/p(3)-1;
toe = 99*exp(3)/(166*exp(3)-67)*p(6);
if strain <= 0
    tendon = 0;
elseif strain < toe
    tendon = 0.33*expm1(3*strain/toe)/expm1(3);
else
    tendon = 0.33+0.67*(strain-toe)/(p(6)-toe);
end
force = p(1)*tendon;
normalizedLength = fiber/p(2);
activeLength = exp(-(normalizedLength-1)^2/p(9));
passive = expm1(p(8)*max(normalizedLength-1,0)/p(7))/expm1(p(8));
a = min(1,max(p(13),activation));
activeIsometric = a*activeLength;
activeForce = tendon/cosPennation-passive;
% Outside the original concentric/eccentric branches, OpenSim extends
% the tangent from its boundary to keep velocity finite.
threshold = p(12)*p(11)*activeIsometric;
edgeForce = min(threshold,max(0,activeForce));
if edgeForce <= activeIsometric
    denom = activeIsometric+edgeForce/p(10);
    deriv = 1/p(10);
else
    scale = (2+2/p(10))/(p(11)-1);
    denom = scale*(activeIsometric*p(11)-edgeForce);
    deriv = -scale;
end
speedScale = 0.25+0.75*a;
edgeSpeed = speedScale*(edgeForce-activeIsometric)/denom;
slope = (speedScale-edgeSpeed*deriv)/denom;
fiberRate = (edgeSpeed+slope*(activeForce-edgeForce))*p(5)*p(2);
if fiberLength <= minFiber && fiberRate < 0
    fiberRate = 0;
end
end
